simulink model "ps5_stage01_openloop_2024a"  (R2024a)
settings: Solver=ode15s  StartTime=0.0  StopTime=1.0  MaxStep=0.001  RelTol=1e-3
settings Model: Creator=tanuj  LastModifiedBy=tanuj
settings DataIOCC: SaveOutput=off

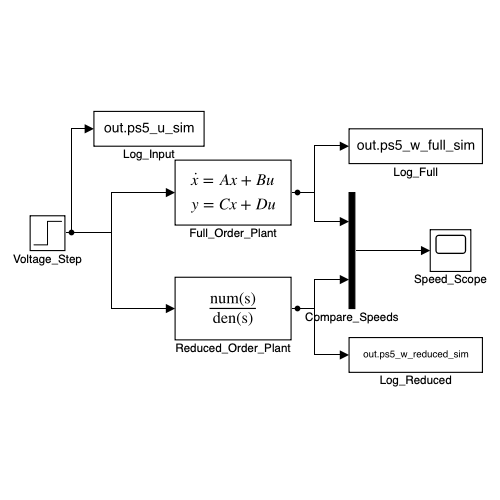
[thumbnail: Simulink's stored preview of the top-level diagram]
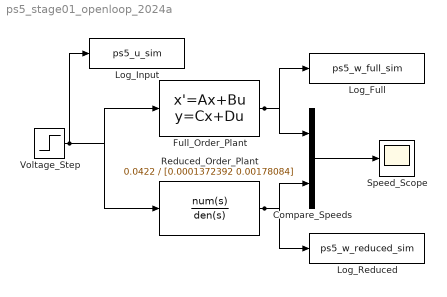
== system ps5_stage01_openloop_2024a ==
  Compare_Speeds : Mux  Inputs=2
  Full_Order_Plant : StateSpace  A=[-6521.739130434783 -36.69565217391305;2306.192399839113 0]  B=[869.5652173913044;0]  C=[0 1]  D=0  InitialCondition=0
  Log_Full : ToWorkspace  VariableName=ps5_w_full_sim  SaveFormat=Timeseries  SampleTime=-1
  Log_Input : ToWorkspace  VariableName=ps5_u_sim  SaveFormat=Timeseries  SampleTime=-1
  Log_Reduced : ToWorkspace  VariableName=ps5_w_reduced_sim  SaveFormat=Timeseries  SampleTime=-1
  Reduced_Order_Plant : TransferFcn  Numerator=0.0422  Denominator=[0.0001372392 0.00178084]
  Speed_Scope : Scope
  Voltage_Step : Step  Time=0.1  After=2  SampleTime=0
  wires:
  Voltage_Step/1 -> Full_Order_Plant/1, Reduced_Order_Plant/1, Log_Input/1
  Full_Order_Plant/1 -> Compare_Speeds/1, Log_Full/1
  Reduced_Order_Plant/1 -> Compare_Speeds/2, Log_Reduced/1
  Compare_Speeds/1 -> Speed_Scope/1
